simulink subsystem "Propellant_Mass_Integration"  (R2026a)
settings: Solver=VariableStepAuto
undefined symbols (not defined in the file): IN
settings Model: Creator=asing  LastModifiedBy=asing

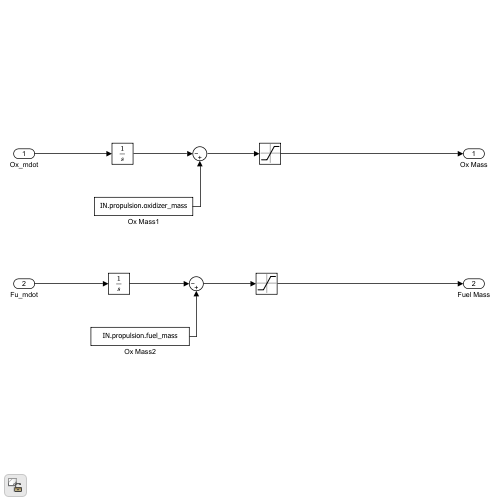
[thumbnail: Simulink's stored preview of the top-level diagram]
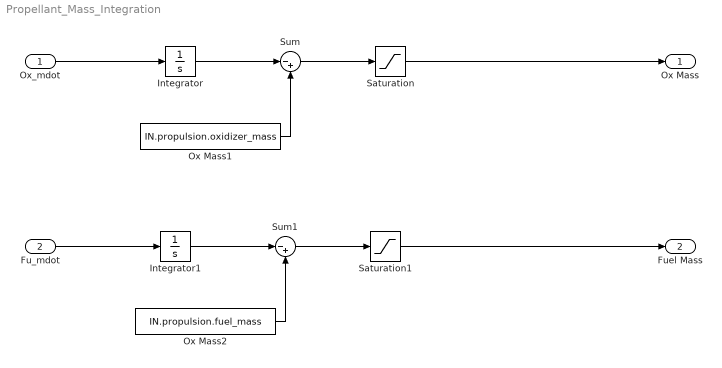
== system Propellant_Mass_Integration ==
  Ox_mdot : Inport
  Fu_mdot : Inport  Port=2
  Integrator : Integrator
  Integrator1 : Integrator
  Ox Mass1 : Constant  Value=IN.propulsion.oxidizer_mass
  Ox Mass2 : Constant  Value=IN.propulsion.fuel_mass
  Saturation : Saturate  UpperLimit=IN.propulsion.oxidizer_mass  LowerLimit=0
  Saturation1 : Saturate  UpperLimit=IN.propulsion.fuel_mass  LowerLimit=0
  Sum : Sum  Inputs=|-+
  Sum1 : Sum  Inputs=|-+
  Ox Mass : Outport
  Fuel Mass : Outport  Port=2
  wires:
  Ox_mdot/1 -> Integrator/1
  Integrator/1 -> Sum/1
  Ox Mass1/1 -> Sum/2
  Sum/1 -> Saturation/1
  Saturation/1 -> Ox Mass/1
  Sum1/1 -> Saturation1/1
  Saturation1/1 -> Fuel Mass/1
  Fu_mdot/1 -> Integrator1/1
  Ox Mass2/1 -> Sum1/2
  Integrator1/1 -> Sum1/1
